simulink model "model"  (R2022b)
settings: Solver=VariableStepAuto  StartTime=0.0  StopTime=10.0  MinStep=1e-10  RelTol=1e-10
values from neighbouring files (symbols this model uses):
  K = 1/ke    (= 3.10366232154)    [parameters.m]
  T = sqrt(Tm*Te)    [parameters.m]
  xi = T/(2*Te)    [parameters.m]
settings Model: Creator=Иван Бакланов  LastModifiedBy=Иван Бакланов

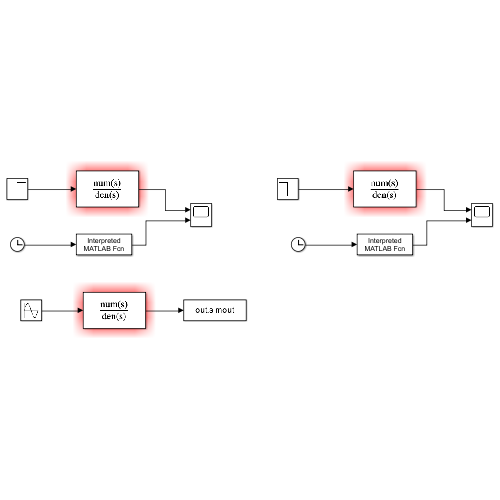
[thumbnail: Simulink's stored preview of the top-level diagram]
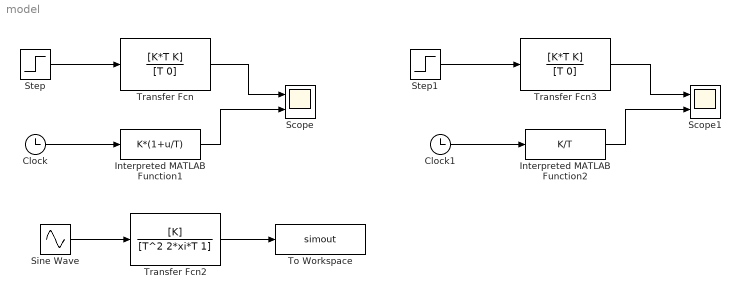
== system model ==
  Clock : Clock
  Clock1 : Clock
  Interpreted MATLAB Function1 : MATLABFcn  MATLABFcn=K*(1+u/T)
  Interpreted MATLAB Function2 : MATLABFcn  MATLABFcn=K/T
  Scope : Scope  NumInputPorts=2
  Scope1 : Scope  NumInputPorts=2
  Sine Wave : Sin  SampleTime=0
  Step : Step  Time=0  SampleTime=0
  Step1 : Step  Time=1e-7  Before=1e7  After=0  SampleTime=0
  To Workspace : ToWorkspace  VariableName=simout  SaveFormat=Timeseries  SampleTime=-1
  Transfer Fcn : TransferFcn  Numerator=[K*T K]  Denominator=[T 0]
  Transfer Fcn2 : TransferFcn  Numerator=[K]  Denominator=[T^2 2*xi*T 1]
  Transfer Fcn3 : TransferFcn  Numerator=[K*T K]  Denominator=[T 0]
  wires:
  Step/1 -> Transfer Fcn/1
  Transfer Fcn/1 -> Scope/1
  Clock/1 -> Interpreted MATLAB Function1/1
  Transfer Fcn3/1 -> Scope1/1
  Interpreted MATLAB Function2/1 -> Scope1/2
  Clock1/1 -> Interpreted MATLAB Function2/1
  Sine Wave/1 -> Transfer Fcn2/1
  Step1/1 -> Transfer Fcn3/1
  Interpreted MATLAB Function1/1 -> Scope/2
  Transfer Fcn2/1 -> To Workspace/1
